simulink model "Test_Model"  (R2024b)
settings: Solver=FixedStepDiscrete  StartTime=0.0  StopTime=0.2  FixedStep=1e-6  RelTol=1e-3
values from neighbouring files (symbols this model uses):
  CHB_MODE : value not decoded    [CHB_Data.sldd]
settings Model: DataDictionary=CHB_Data.sldd  PauseTimes=0.  Creator=licuiting  LastModifiedBy=licuiting
settings DataIOCC: ReturnWorkspaceOutputs=off

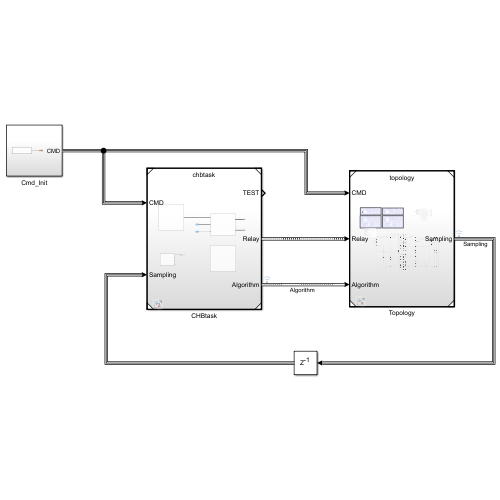
[thumbnail: Simulink's stored preview of the top-level diagram]
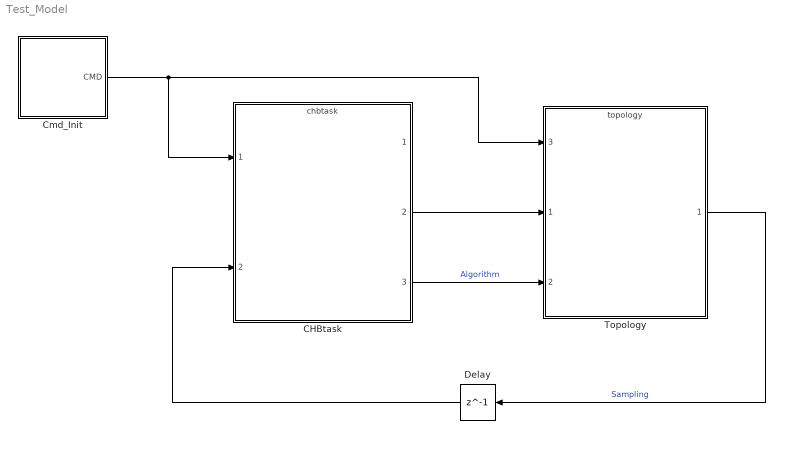
== system Test_Model ==
  CHBtask : ModelReference  ModelNameDialog=chbtask.slx  SimulationMode=Normal  ModelReferenceVersion=1.93
  Cmd_Init : Subsystem
  Delay : Delay  DelayLength=1  InputProcessing=Columns as channels (frame based)
  Topology : ModelReference  ModelNameDialog=topology.slx  SimulationMode=Normal  ModelReferenceVersion=1.58
      settings: PortSchema="{\"entries\":[{\"content\":{\"sides\":[{\"content\":{\"connectorIds\":[\"In3\",\"In1\",\"In2\"]},\"type\":\"ConnectorPlacement.EquallySpacedRectSide\",\"uuid\":\"ea2f3b83-6769-4991-9c1c-b90b49d748ed\"},{\"content\":{\"connectorIds\":[\"Out1\"],\"side\":\"RIGHT\"},\"type\":\"ConnectorPlacement.EquallySpacedRectSide\",\"uuid\":\"0ff6ed6a-c596-4816-bfbe-7829c8e49149\"},{\"content\":{\"side\":\"TOP\"},\"type\":\"ConnectorPlacement.EquallySpacedRectSide\",\"uuid\":\"a4032569-4e2e-43b8-a863-f6d95e409479\"}]},\"type\":\"ConnectorPlacement.EquallySpacedConnector\",\"uuid\":\"30aad47c-d2c2-490c-acce-f147a2aecd98\"}],\"packageUris\":[\"http://schema.mathworks.com/mf0/Connector/R2020b\"],\"version\":\"1.0\"}"
  wires:
  Topology/1 -> Delay/1  "Sampling"
  Delay/1 -> CHBtask/2
  CHBtask/2 -> Topology/1
  CHBtask/3 -> Topology/2  "Algorithm"
  Cmd_Init/1(CMD) -> CHBtask/1, Topology/3

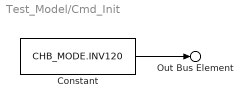
== system Test_Model/Cmd_Init ==
  Constant : Constant  Value=CHB_MODE.INV120  OutDataTypeStr=Enum: CHB_MODE
  Out Bus Element : Outport  PortName=CMD  Element=run_model
  wires:
  Constant/1 -> Out Bus Element/1
